simulink model "InductionHeating_bb_4"  (R2026b)
settings: Solver=FixedStepDiscrete  StopTime=0.008
PostLoadFcn:
  | Ts = 1e-6;Ts_fpga=10e-9;   R=3; Capa=300e-9;L=100e-6;Pejo_factor=1;
InitFcn:
  | Ts = 1e-6;Ts_fpga=10e-9;   R=3; Capa=300e-9;L=100e-6;Pejo_factor=1;
undefined symbols (not defined in the file or in its folder): DiscIntNeverNeededParam, ee_sli_rtmsupport, gcbh, isSetWhenUndefinedState, MATESOCwDio
libraries: fl_lib x67, nesl_utility x40, hdlsllib x32, simulink x15, eeGeneralControl x9, ee_lib x3
(part 6 of 7)

== system InductionHeating_bb_4/soc16/DynamicMultMAT/add2 ==
  E : Inport
  In1 : Inport  Port=2
  In2 : Inport  Port=3
  In4 : Inport  Port=4
  In5 : Inport  Port=5
  In7 : Inport  Port=6
  In8 : Inport  Port=7
  In10 : Inport  Port=8
  In11 : Inport  Port=9
  Add{3..6} (4 alike) : Sum
  Unit Delay Enabled Synchronous{1..3,22} (4 alike) : hdlsllib/Discrete/Unit Delay Enabled Synchronous  InitialCondition=0.0  SampleTime=-1
  y : Outport
  y1 : Outport  Port=2
  y2 : Outport  Port=3
  y3 : Outport  Port=4
  wires:
  In11/1 -> Add6/2
  In7/1 -> Add5/1
  Unit Delay Enabled Synchronous22/1 -> y/1
  Unit Delay Enabled Synchronous2/1 -> y2/1
  In10/1 -> Add6/1
  In2/1 -> Add3/2
  In8/1 -> Add5/2
  In4/1 -> Add4/1
  E/1 -> Unit Delay Enabled Synchronous22/2, Unit Delay Enabled Synchronous1/2, Unit Delay Enabled Synchronous2/2, Unit Delay Enabled Synchronous3/2
  Unit Delay Enabled Synchronous3/1 -> y3/1
  Unit Delay Enabled Synchronous1/1 -> y1/1
  Add5/1 -> Unit Delay Enabled Synchronous2/1
  Add3/1 -> Unit Delay Enabled Synchronous22/1
  Add6/1 -> Unit Delay Enabled Synchronous3/1
  In5/1 -> Add4/2
  In1/1 -> Add3/1
  Add4/1 -> Unit Delay Enabled Synchronous1/1

== system InductionHeating_bb_4/soc16/DynamicMultMAT/add3 ==
  E : Inport
  In1 : Inport  Port=2
  In2 : Inport  Port=3
  In4 : Inport  Port=4
  In5 : Inport  Port=5
  In7 : Inport  Port=6
  In8 : Inport  Port=7
  In10 : Inport  Port=8
  In11 : Inport  Port=9
  Add{3..6} (4 alike) : Sum
  Unit Delay Enabled Synchronous{1..3,22} (4 alike) : hdlsllib/Discrete/Unit Delay Enabled Synchronous  InitialCondition=0.0  SampleTime=-1
  y : Outport
  y1 : Outport  Port=2
  y2 : Outport  Port=3
  y3 : Outport  Port=4
  wires:
  Add4/1 -> Unit Delay Enabled Synchronous1/1
  In1/1 -> Add3/1
  In5/1 -> Add4/2
  Add6/1 -> Unit Delay Enabled Synchronous3/1
  Add3/1 -> Unit Delay Enabled Synchronous22/1
  Add5/1 -> Unit Delay Enabled Synchronous2/1
  Unit Delay Enabled Synchronous1/1 -> y1/1
  Unit Delay Enabled Synchronous3/1 -> y3/1
  E/1 -> Unit Delay Enabled Synchronous3/2, Unit Delay Enabled Synchronous2/2, Unit Delay Enabled Synchronous1/2, Unit Delay Enabled Synchronous22/2
  In4/1 -> Add4/1
  In8/1 -> Add5/2
  In2/1 -> Add3/2
  In10/1 -> Add6/1
  Unit Delay Enabled Synchronous2/1 -> y2/1
  Unit Delay Enabled Synchronous22/1 -> y/1
  In7/1 -> Add5/1
  In11/1 -> Add6/2

== system InductionHeating_bb_4/soc16/DynamicMultMAT/add4 ==
  E : Inport
  In1 : Inport  Port=2
  In2 : Inport  Port=3
  In4 : Inport  Port=4
  In5 : Inport  Port=5
  In7 : Inport  Port=6
  In8 : Inport  Port=7
  In10 : Inport  Port=8
  In11 : Inport  Port=9
  Add{3..6} (4 alike) : Sum
  Unit Delay Enabled Synchronous{1..3,22} (4 alike) : hdlsllib/Discrete/Unit Delay Enabled Synchronous  InitialCondition=0.0  SampleTime=-1
  y : Outport
  y1 : Outport  Port=2
  y2 : Outport  Port=3
  y3 : Outport  Port=4
  wires:
  In11/1 -> Add6/2
  In7/1 -> Add5/1
  Unit Delay Enabled Synchronous22/1 -> y/1
  Unit Delay Enabled Synchronous2/1 -> y2/1
  In10/1 -> Add6/1
  In2/1 -> Add3/2
  In8/1 -> Add5/2
  In4/1 -> Add4/1
  E/1 -> Unit Delay Enabled Synchronous22/2, Unit Delay Enabled Synchronous1/2, Unit Delay Enabled Synchronous2/2, Unit Delay Enabled Synchronous3/2
  Unit Delay Enabled Synchronous3/1 -> y3/1
  Unit Delay Enabled Synchronous1/1 -> y1/1
  Add5/1 -> Unit Delay Enabled Synchronous2/1
  Add3/1 -> Unit Delay Enabled Synchronous22/1
  Add6/1 -> Unit Delay Enabled Synchronous3/1
  In5/1 -> Add4/2
  In1/1 -> Add3/1
  Add4/1 -> Unit Delay Enabled Synchronous1/1

== system InductionHeating_bb_4/soc16/DynamicMultMAT/dot1 ==
  note: dot1
  In1 : Inport
  In2 : Inport  Port=2
  In3 : Inport  Port=3
  In4 : Inport  Port=4
  In5 : Inport  Port=5
  In6 : Inport  Port=6
  In7 : Inport  Port=7
  In8 : Inport  Port=8
  Dot Product{,1..3} (4 alike) : DotProduct  OutDataTypeStr=Inherit: Inherit via internal rule
  Out1 : Outport
  Out2 : Outport  Port=2
  Out3 : Outport  Port=3
  Out4 : Outport  Port=4
  wires:
  In1/1 -> Dot Product/2
  Dot Product/1 -> Out1/1
  In3/1 -> Dot Product1/2
  Dot Product1/1 -> Out2/1
  In2/1 -> Dot Product/1
  Dot Product3/1 -> Out4/1
  Dot Product2/1 -> Out3/1
  In7/1 -> Dot Product3/2
  In5/1 -> Dot Product2/2
  In8/1 -> Dot Product3/1
  In4/1 -> Dot Product1/1
  In6/1 -> Dot Product2/1

== system InductionHeating_bb_4/soc16/DynamicMultMAT/dot2 ==
  In1 : Inport
  y : Inport  Port=2
  In3 : Inport  Port=3
  y1 : Inport  Port=4
  In5 : Inport  Port=5
  y2 : Inport  Port=6
  In7 : Inport  Port=7
  y3 : Inport  Port=8
  Dot Product{4..7} (4 alike) : DotProduct  OutDataTypeStr=Inherit: Inherit via internal rule
  Out1 : Outport
  Out2 : Outport  Port=2
  Out3 : Outport  Port=3
  Out4 : Outport  Port=4
  wires:
  In3/1 -> Dot Product5/2
  Dot Product7/1 -> Out4/1
  Dot Product4/1 -> Out1/1
  Dot Product6/1 -> Out3/1
  In1/1 -> Dot Product4/2
  In7/1 -> Dot Product7/2
  Dot Product5/1 -> Out2/1
  In5/1 -> Dot Product6/2
  y/1 -> Dot Product4/1
  y1/1 -> Dot Product5/1
  y2/1 -> Dot Product6/1
  y3/1 -> Dot Product7/1

== system InductionHeating_bb_4/soc16/DynamicMultMAT/dot3 ==
  In1 : Inport
  y : Inport  Port=2
  In3 : Inport  Port=3
  y1 : Inport  Port=4
  In5 : Inport  Port=5
  y2 : Inport  Port=6
  In7 : Inport  Port=7
  y3 : Inport  Port=8
  Dot Product{8..11} (4 alike) : DotProduct  OutDataTypeStr=Inherit: Inherit via internal rule
  Out1 : Outport
  Out2 : Outport  Port=2
  Out3 : Outport  Port=3
  Out4 : Outport  Port=4
  wires:
  Dot Product11/1 -> Out4/1
  Dot Product10/1 -> Out3/1
  Dot Product8/1 -> Out1/1
  Dot Product9/1 -> Out2/1
  In3/1 -> Dot Product9/2
  In5/1 -> Dot Product10/2
  In7/1 -> Dot Product11/2
  In1/1 -> Dot Product8/2
  y3/1 -> Dot Product11/1
  y2/1 -> Dot Product10/1
  y/1 -> Dot Product8/1
  y1/1 -> Dot Product9/1

== system InductionHeating_bb_4/soc16/DynamicMultMAT/dot4 ==
  In1 : Inport
  In2 : Inport  Port=2
  In3 : Inport  Port=3
  In4 : Inport  Port=4
  In5 : Inport  Port=5
  Dot Product{12..15} (4 alike) : DotProduct  OutDataTypeStr=Inherit: Inherit via internal rule
  Out1 : Outport
  Out2 : Outport  Port=2
  Out3 : Outport  Port=3
  Out4 : Outport  Port=4
  wires:
  In1/1 -> Dot Product15/2, Dot Product14/2, Dot Product13/2, Dot Product12/2
  Dot Product14/1 -> Out3/1
  In5/1 -> Dot Product15/1
  In3/1 -> Dot Product13/1
  Dot Product15/1 -> Out4/1
  Dot Product13/1 -> Out2/1
  Dot Product12/1 -> Out1/1
  In2/1 -> Dot Product12/1
  In4/1 -> Dot Product14/1

== system InductionHeating_bb_4/soc16/DynamicMultMAT/mult1 ==
  In1 : Inport
  In2 : Inport  Port=2
  In3 : Inport  Port=3
  In4 : Inport  Port=4
  In5 : Inport  Port=5
  In6 : Inport  Port=6
  In7 : Inport  Port=7
  In8 : Inport  Port=8
  mullt{1..4} (4 alike) : Product
  DxCol*DxRow : Outport
  DxCol*DxRow1 : Outport  Port=2
  DxCol*DxRow2 : Outport  Port=3
  DxCol*DxRow3 : Outport  Port=4
  wires:
  mullt4/1 -> DxCol*DxRow3/1  "DxCol*DxRow"
  In2/1 -> mullt1/2
  In4/1 -> mullt2/2
  mullt2/1 -> DxCol*DxRow1/1  "DxCol*DxRow"
  In1/1 -> mullt1/1
  In8/1 -> mullt4/2
  In3/1 -> mullt2/1
  In6/1 -> mullt3/2
  In7/1 -> mullt4/1
  mullt1/1 -> DxCol*DxRow/1  "DxCol*DxRow"
  mullt3/1 -> DxCol*DxRow2/1  "DxCol*DxRow"
  In5/1 -> mullt3/1

== system InductionHeating_bb_4/soc16/DynamicMultMAT/mult2 ==
  In1 : Inport
  In2 : Inport  Port=2
  In3 : Inport  Port=3
  In4 : Inport  Port=4
  In5 : Inport  Port=5
  In6 : Inport  Port=6
  In7 : Inport  Port=7
  In8 : Inport  Port=8
  mullt{1..4} (4 alike) : Product
  DxCol*DxRow : Outport
  DxCol*DxRow1 : Outport  Port=2
  DxCol*DxRow2 : Outport  Port=3
  DxCol*DxRow3 : Outport  Port=4
  wires:
  In5/1 -> mullt3/1
  mullt3/1 -> DxCol*DxRow2/1  "DxCol*DxRow"
  mullt1/1 -> DxCol*DxRow/1  "DxCol*DxRow"
  In7/1 -> mullt4/1
  In6/1 -> mullt3/2
  In3/1 -> mullt2/1
  In8/1 -> mullt4/2
  In1/1 -> mullt1/1
  mullt2/1 -> DxCol*DxRow1/1  "DxCol*DxRow"
  In4/1 -> mullt2/2
  In2/1 -> mullt1/2
  mullt4/1 -> DxCol*DxRow3/1  "DxCol*DxRow"

== system InductionHeating_bb_4/soc16/DynamicMultMAT/mult3 ==
  In1 : Inport
  In2 : Inport  Port=2
  In3 : Inport  Port=3
  In4 : Inport  Port=4
  In5 : Inport  Port=5
  In6 : Inport  Port=6
  In7 : Inport  Port=7
  In8 : Inport  Port=8
  mullt{1..4} (4 alike) : Product
  DxCol*DxRow : Outport
  DxCol*DxRow1 : Outport  Port=2
  DxCol*DxRow2 : Outport  Port=3
  DxCol*DxRow3 : Outport  Port=4
  wires:
  mullt4/1 -> DxCol*DxRow3/1  "DxCol*DxRow"
  In2/1 -> mullt1/2
  In4/1 -> mullt2/2
  mullt2/1 -> DxCol*DxRow1/1  "DxCol*DxRow"
  In1/1 -> mullt1/1
  In8/1 -> mullt4/2
  In3/1 -> mullt2/1
  In6/1 -> mullt3/2
  In7/1 -> mullt4/1
  mullt1/1 -> DxCol*DxRow/1  "DxCol*DxRow"
  mullt3/1 -> DxCol*DxRow2/1  "DxCol*DxRow"
  In5/1 -> mullt3/1

== system InductionHeating_bb_4/soc16/DynamicMultMAT/mult4 ==
  In1 : Inport
  In2 : Inport  Port=2
  In3 : Inport  Port=3
  In4 : Inport  Port=4
  In5 : Inport  Port=5
  In6 : Inport  Port=6
  In7 : Inport  Port=7
  In8 : Inport  Port=8
  mullt{1..4} (4 alike) : Product
  DxCol*DxRow : Outport
  DxCol*DxRow1 : Outport  Port=2
  DxCol*DxRow2 : Outport  Port=3
  DxCol*DxRow3 : Outport  Port=4
  wires:
  In5/1 -> mullt3/1
  mullt3/1 -> DxCol*DxRow2/1  "DxCol*DxRow"
  mullt1/1 -> DxCol*DxRow/1  "DxCol*DxRow"
  In7/1 -> mullt4/1
  In6/1 -> mullt3/2
  In3/1 -> mullt2/1
  In8/1 -> mullt4/2
  In1/1 -> mullt1/1
  mullt2/1 -> DxCol*DxRow1/1  "DxCol*DxRow"
  In4/1 -> mullt2/2
  In2/1 -> mullt1/2
  mullt4/1 -> DxCol*DxRow3/1  "DxCol*DxRow"

== system InductionHeating_bb_4/soc16/DynamicMultMAT/multdiv1 ==
  In1 : Inport
  In2 : Inport  Port=2
  Demux : Demux  Outputs=[8 8]
  Divide5 : Product  Commented=on
  Mux : Mux  Inputs=2
  mmul8_1 : Subsystem
      mask help: To split one 1x8 vector multiplication
      mask Display: disp('1X8')
  mmul8_11 : Subsystem
      mask help: To split one 1x8 vector multiplication
      mask Display: disp('1X8')
  DxCol_ : Outport
  wires:
  In1/1 -> mmul8_1/1(In1), mmul8_11/1(In1), Divide5/1
  Demux/1 -> mmul8_11/2(In2)
  Demux/2 -> mmul8_1/2(In2)
  In2/1 -> Demux/1
  mmul8_11/1(Out1) -> Mux/1
  mmul8_1/1(Out1) -> Mux/2
  Mux/1 -> DxCol_/1

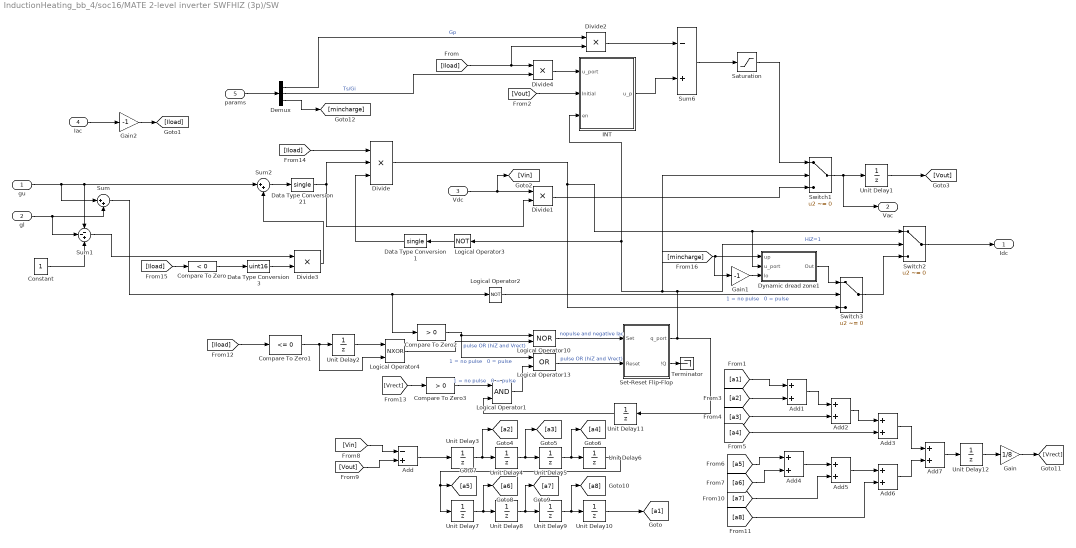
== system InductionHeating_bb_4/soc16/MATE 2-level inverter SWFHIZ (3p)/SW ==
  gu : Inport
  gl : Inport  Port=2
  Vdc : Inport  Port=3
  Iac : Inport  Port=4
  params : Inport  Port=5
  Add : Sum  Inputs=-+
  Add{1..7} (7 alike) : Sum  Inputs=2
  Compare To Zero : simulink/Logic and Bit Operations/Compare To Zero  relop=<  OutDataTypeStr=boolean
  Compare To Zero1 : simulink/Logic and Bit Operations/Compare To Zero  relop=<=  OutDataTypeStr=boolean
  Compare To Zero2 : simulink/Logic and Bit Operations/Compare To Zero  relop=>  OutDataTypeStr=boolean
  Compare To Zero3 : simulink/Logic and Bit Operations/Compare To Zero  relop=>  OutDataTypeStr=boolean
  Constant : Constant  OutDataTypeStr=uint16  SampleTime=Ts
  Data Type Conversion1 : DataTypeConversion  OutDataTypeStr=single  RndMeth=Nearest  SaturateOnIntegerOverflow=off
  Data Type Conversion21 : DataTypeConversion  OutDataTypeStr=single  RndMeth=Nearest  SaturateOnIntegerOverflow=off
  Data Type Conversion3 : DataTypeConversion  OutDataTypeStr=uint16  RndMeth=Nearest  SaturateOnIntegerOverflow=off
  Demux : Demux  Outputs=[1 1 1]
  Divide : Product  Inputs=3
  Divide{1..4} (4 alike) : Product
  Dynamic dread zone1 : Subsystem
  Gain : Gain  Gain=1/8
  Gain1 : Gain  Gain=-1
  Gain2 : Gain  Gain=-1
  INT : Subsystem
  Logical Operator1 : Logic  AllPortsSameDT=off  OutDataTypeStr=boolean
  Logical Operator10 : Logic  Operator=NOR  AllPortsSameDT=off  OutDataTypeStr=boolean
  Logical Operator13 : Logic  Operator=OR  AllPortsSameDT=off  OutDataTypeStr=boolean
  Logical Operator2 : Logic  Operator=NOT  AllPortsSameDT=off  OutDataTypeStr=boolean
  Logical Operator3 : Logic  Operator=NOT  AllPortsSameDT=off  OutDataTypeStr=boolean
  Logical Operator4 : Logic  Operator=NXOR  AllPortsSameDT=off  OutDataTypeStr=boolean
  Saturation : Saturate  UpperLimit=inf  LowerLimit=0
  Set-Reset Flip-Flop : Subsystem  AncestorBlock=eeGeneralControl/Set-Reset Flip-Flop  LoadFcn=ee_sli_rtmsupport( 'loadfcn', gcbh );  Variant=on  VariantControlMode=label  LabelModeActiveChoice=Discrete  mask(Set-Reset Flip-Flop){UndefState=Set, Q0=0, Ts=Ts}
      mask prompts: UndefState "physmod:ee:library:comments:control:eeGeneralControl:PriorityWhenUndefinedState_MP"; Q0 "physmod:ee:library:comments:control:eeGeneralControl:InitialConditionForQState_MP"; Ts "physmod:ee:library:comments:control:eeGeneralControl:SampleTime1ForInherited_MP"
      mask help: physmod:ee:library:comments:control:eeGeneralControl:SetResetFlipFlop_MD
      mask init:
      | [timeDomain,isSetWhenUndefinedState] = ee.mask.initializeSetResetFlipFlop(gcb,Q0,Ts,UndefState);%#ok
      settings: CopyFcn=ee_sli_rtmsupport( 'copyfcn', gcbh );  DeleteFcn=ee_sli_rtmsupport( 'deletefcn', gcbh );  ModelCloseFcn=ee_sli_rtmsupport( 'modelclosefcn', gcbh );  PostSaveFcn=ee_sli_rtmsupport( 'postsavefcn', gcbh );  PreCopyFcn=ee_sli_rtmsupport( 'precopyfcn', gcbh );  OpenFcn=ee_sli_rtmsupport( 'openfcn', gcbh );  CloseFcn=ee_sli_rtmsupport( 'closefcn', gcbh );  PreDeleteFcn=ee_sli_rtmsupport( 'predeletefcn', gcbh );
      mask Help: web(nesl_help(gcbh))
      mask TypeOptions UndefState: physmod:ee:library:comments:control:eeGeneralControl:Reset_PV | physmod:ee:library:comments:control:eeGeneralControl:Set_PV
      mask DialogControl ParameterGroupVar Prompt: physmod:ee:library:comments:control:eeGeneralControl:tab_Parameters
      mask DialogControl UndefState Prompt: Priority when undefined state
      mask DialogControl Q0 Prompt: Initial condition for Q state
      mask DialogControl Ts Prompt: Sample time (-1 for inherited)
      mask Display: ee.mask.drawSetResetFlipFlop;
  Sum : Sum  Inputs=|++
  Sum1 : Sum  Inputs=--+
  Sum2 : Sum  Inputs=|++
  Sum6 : Sum  Inputs=-+  InputSameDT=on  SaturateOnIntegerOverflow=on  SampleTime=Ts  OutDataTypeStr=Inherit: Same as first input
  Switch1 : Switch  Criteria=u2 ~= 0  SaturateOnIntegerOverflow=off  InputSameDT=off
  Switch2 : Switch  Criteria=u2 ~= 0  Threshold=0.5  SaturateOnIntegerOverflow=off  InputSameDT=off
  Switch3 : Switch  Criteria=u2 ~= 0  Threshold=0.5  SaturateOnIntegerOverflow=off  InputSameDT=off
  Terminator : Terminator
  Unit Delay{1..12} (12 alike) : UnitDelay  SampleTime=Ts
  Idc : Outport  VectorParamsAs1DForOutWhenUnconnected=off
  Vac : Outport  Port=2  VectorParamsAs1DForOutWhenUnconnected=off
  wires:
  Set-Reset Flip-Flop/2(!Q) -> Terminator/1
  Iac/1 -> Gain2/1
  Set-Reset Flip-Flop/1(q_port) -> Logical Operator3/1, INT/3(en), Switch1/2, Switch2/2, Unit Delay11/1  "HiZ=1"
  Sum6/1 -> Saturation/1
  Switch1/1 -> Unit Delay1/1, Vac/1
  Constant/1 -> Sum1/3
  gl/1 -> Sum1/2, Sum/2
  Logical Operator3/1 -> Data Type Conversion1/1
  Logical Operator2/1 -> Switch3/2  "1 = no pulse   0 = pulse"
  Vdc/1 -> Divide1/1, [Vin]
  Sum/1 -> Logical Operator2/1, Compare To Zero2/1
  gu/1 -> Sum/1, Sum2/1, Sum1/1
  Sum2/1 -> Data Type Conversion21/1
  Divide1/1 -> Switch1/3
  Saturation/1 -> Switch1/1
  Switch2/1 -> Idc/1
  Divide/1 -> Switch3/3, Dynamic dread zone1/2(u_port), Switch2/1
  Dynamic dread zone1/1(Out) -> Switch3/1
  Switch3/1 -> Switch2/3
  Unit Delay1/1 -> [Vout]
  Logical Operator10/1 -> Set-Reset Flip-Flop/1(Set)  "nopulse and negative Iac"
  [Vout] -> INT/2(Initial)
  [Vin] -> Add/1
  [Vout] -> Add/2
  Add/1 -> Unit Delay3/1
  Unit Delay3/1 -> [a2], Unit Delay4/1
  Unit Delay4/1 -> [a3], Unit Delay5/1
  Unit Delay5/1 -> [a4], Unit Delay6/1
  Unit Delay6/1 -> [a5], Unit Delay7/1
  Unit Delay7/1 -> [a6], Unit Delay8/1
  Unit Delay8/1 -> [a7], Unit Delay9/1
  Unit Delay9/1 -> Unit Delay10/1, [a8]
  [a4] -> Add3/2
  [a3] -> Add2/2
  [a2] -> Add1/2
  [a1] -> Add1/1
  Compare To Zero1/1 -> Logical Operator4/2, Unit Delay2/1
  INT/1(u_p) -> Sum6/2
  [Vrect] -> Compare To Zero3/1
  Unit Delay11/1 -> Logical Operator1/2
  Logical Operator13/1 -> Set-Reset Flip-Flop/2(Reset)  "pulse OR (hiZ and Vrect)"
  Logical Operator1/1 -> Logical Operator13/2
  [Iload] -> Divide4/1, Divide2/2
  [Iload] -> Divide/1
  [Iload] -> Compare To Zero/1
  Compare To Zero/1 -> Data Type Conversion3/1
  Sum1/1 -> Divide3/1
  Gain2/1 -> [Iload]
  Demux/1 -> Divide2/1  "Gp"
  Divide2/1 -> Sum6/1
  Divide4/1 -> INT/1(u_port)
  Demux/2 -> Divide4/2  "Ts/Gi"
  Demux/3 -> [mincharge]
  [mincharge] -> Dynamic dread zone1/1(up), Gain1/1
  Gain1/1 -> Dynamic dread zone1/3(lo)
  params/1 -> Demux/1
  Data Type Conversion21/1 -> Divide1/2, Divide/2
  Data Type Conversion1/1 -> Divide/3
  Gain/1 -> [Vrect]
  [a5] -> Add4/1
  [a6] -> Add4/2
  [a7] -> Add5/2
  [a8] -> Add6/2
  Add1/1 -> Add2/1
  Add2/1 -> Add3/1
  Add4/1 -> Add5/1
  Add5/1 -> Add6/1
  Add3/1 -> Add7/1
  Add6/1 -> Add7/2
  Add7/1 -> Unit Delay12/1
  Divide3/1 -> Sum2/2
  Data Type Conversion3/1 -> Divide3/2
  Unit Delay2/1 -> Logical Operator4/1
  Logical Operator4/1 -> Logical Operator10/2  "pulse OR (hiZ and Vrect)"
  Compare To Zero2/1 -> Logical Operator10/1, Logical Operator13/1  "1 = no pulse   0 = pulse"
  Unit Delay10/1 -> [a1]
  Compare To Zero3/1 -> Logical Operator1/1  "1 = no pulse   0 = pulse"
  [Iload] -> Compare To Zero1/1
  Unit Delay12/1 -> Gain/1

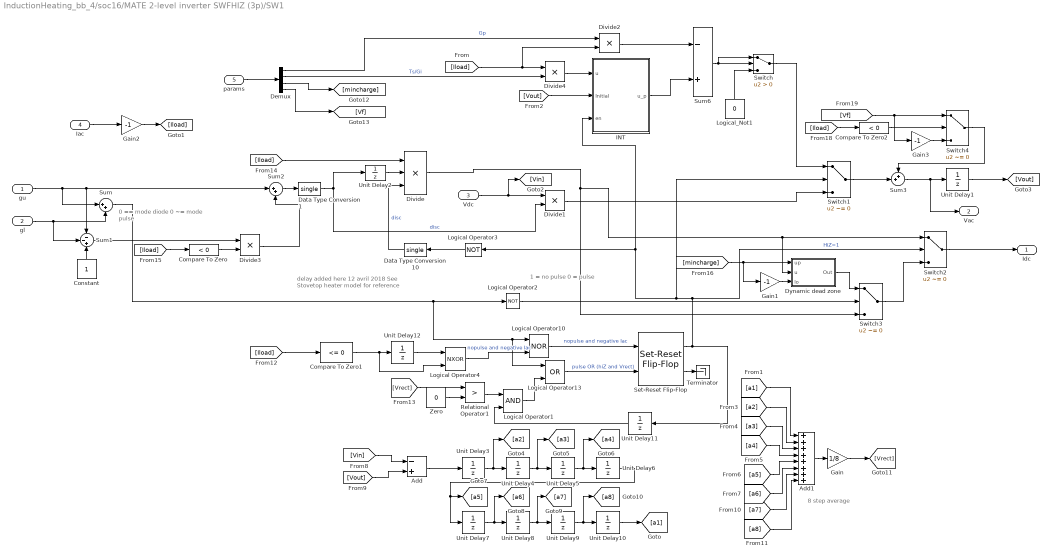
== system InductionHeating_bb_4/soc16/MATE 2-level inverter SWFHIZ (3p)/SW1 ==
  note: 8 step average
  note: 1 = no pulse
      | 0 = pulse
  note: 0 == mode diode
      | 0 ~= mode pulse
  note: delay added here 12 avril 2018
      | See Stovetop heater model for reference
  gu : Inport
  gl : Inport  Port=2
  Vdc : Inport  Port=3
  Iac : Inport  Port=4
  params : Inport  Port=5
  Add : Sum  Inputs=-+
  Add1 : Sum  Inputs=8
  Compare To Zero : simulink/Logic and Bit Operations/Compare To Zero  relop=<  OutDataTypeStr=boolean
  Compare To Zero1 : simulink/Logic and Bit Operations/Compare To Zero  relop=<=  OutDataTypeStr=boolean
  Compare To Zero2 : simulink/Logic and Bit Operations/Compare To Zero  relop=<  OutDataTypeStr=boolean
  Constant : Constant  OutDataTypeStr=uint16
  Data Type Conversion1 : DataTypeConversion  OutDataTypeStr=single  RndMeth=Nearest  SaturateOnIntegerOverflow=off
  Data Type Conversion10 : DataTypeConversion  OutDataTypeStr=single  RndMeth=Nearest  SaturateOnIntegerOverflow=off
  Demux : Demux
  Divide : Product  Inputs=3
  Divide{1..4} (4 alike) : Product
  Dynamic dead zone : Subsystem
  Gain : Gain  Gain=1/8
  Gain1 : Gain  Gain=-1
  Gain2 : Gain  Gain=-1
  Gain3 : Gain  Gain=-1
  INT : Subsystem
  Logical Operator1 : Logic  AllPortsSameDT=off  OutDataTypeStr=boolean
  Logical Operator10 : Logic  Operator=NOR  AllPortsSameDT=off  OutDataTypeStr=boolean
  Logical Operator13 : Logic  Operator=OR  AllPortsSameDT=off  OutDataTypeStr=boolean
  Logical Operator2 : Logic  Operator=NOT  AllPortsSameDT=off  OutDataTypeStr=boolean
  Logical Operator3 : Logic  Operator=NOT  AllPortsSameDT=off  OutDataTypeStr=boolean
  Logical Operator4 : Logic  Operator=NXOR  AllPortsSameDT=off  OutDataTypeStr=boolean
  Logical_Not1 : Constant  Value=0  OutDataTypeStr=single  SampleTime=-1
  Relational Operator1 : RelationalOperator  Operator=>  OutDataTypeStr=boolean  InputSameDT=off
  Set-Reset Flip-Flop : eeGeneralControl/Set-Reset Flip-Flop  LabelModeActiveChoice=Discrete  UndefState=Set  Q0=0  Ts=Ts
  Sum : Sum  Inputs=|++
  Sum1 : Sum  Inputs=--+
  Sum2 : Sum  Inputs=|++
  Sum3 : Sum  Inputs=++|
  Sum6 : Sum  Inputs=-+  InputSameDT=on  SaturateOnIntegerOverflow=on  SampleTime=Ts  OutDataTypeStr=Inherit: Same as first input
  Switch : Switch  Criteria=u2 > Threshold  SaturateOnIntegerOverflow=off  InputSameDT=off
  Switch1 : Switch  Criteria=u2 ~= 0  SaturateOnIntegerOverflow=off  InputSameDT=off
  Switch2 : Switch  Criteria=u2 ~= 0  Threshold=0.5  SaturateOnIntegerOverflow=off  InputSameDT=off
  Switch3 : Switch  Criteria=u2 ~= 0  Threshold=0.5  SaturateOnIntegerOverflow=off  InputSameDT=off
  Switch4 : Switch  Criteria=u2 ~= 0  Threshold=0.5  SaturateOnIntegerOverflow=off  InputSameDT=off
  Terminator : Terminator
  Unit Delay{1..12} (12 alike) : UnitDelay  SampleTime=Ts
  Zero : Constant  Value=0  OutDataTypeStr=single
  Idc : Outport  VectorParamsAs1DForOutWhenUnconnected=off
  Vac : Outport  Port=2  VectorParamsAs1DForOutWhenUnconnected=off
  wires:
  Logical Operator4/1 -> Logical Operator10/2  "nopulse and negative Iac"
  Unit Delay12/1 -> Logical Operator4/1
  Unit Delay10/1 -> [a1]
  Unit Delay2/1 -> Divide/2
  Switch4/1 -> Sum3/1
  Gain3/1 -> Switch4/3
  [Vf] -> Switch4/1, Gain3/1
  Compare To Zero2/1 -> Switch4/2
  Sum3/1 -> Vac/1, Unit Delay1/1
  [Iload] -> Compare To Zero2/1
  Demux/4 -> [Vf]
  params/1 -> Demux/1
  Gain1/1 -> Dynamic dead zone/3(lo)
  [mincharge] -> Gain1/1, Dynamic dead zone/1(up)
  Demux/3 -> [mincharge]
  Demux/2 -> Divide4/2  "Ts/Gi"
  Divide4/1 -> INT/1(u)
  Divide2/1 -> Sum6/1
  Demux/1 -> Divide2/1  "Gp"
  Gain2/1 -> [Iload]
  Sum1/1 -> Divide3/1
  Compare To Zero/1 -> Divide3/2
  [Iload] -> Compare To Zero/1
  [Iload] -> Divide/1
  [Iload] -> Divide2/2, Divide4/1
  Logical Operator1/1 -> Logical Operator13/2
  Logical Operator13/1 -> Set-Reset Flip-Flop/2  "pulse OR (hiZ and Vrect)"
  Unit Delay11/1 -> Logical Operator1/2
  Relational Operator1/1 -> Logical Operator1/1
  Zero/1 -> Relational Operator1/2
  [Vrect] -> Relational Operator1/1
  INT/1(u_p) -> Sum6/2
  Compare To Zero1/1 -> Unit Delay12/1, Logical Operator4/2
  [Iload] -> Compare To Zero1/1
  Gain/1 -> [Vrect]
  Add1/1 -> Gain/1
  [a1] -> Add1/1
  [a8] -> Add1/8
  [a2] -> Add1/2
  [a7] -> Add1/7
  [a6] -> Add1/6
  [a3] -> Add1/3
  [a5] -> Add1/5
  [a4] -> Add1/4
  Unit Delay9/1 -> Unit Delay10/1, [a8]
  Unit Delay8/1 -> Unit Delay9/1, [a7]
  Unit Delay7/1 -> Unit Delay8/1, [a6]
  Unit Delay6/1 -> Unit Delay7/1, [a5]
  Unit Delay5/1 -> Unit Delay6/1, [a4]
  Unit Delay4/1 -> Unit Delay5/1, [a3]
  Unit Delay3/1 -> Unit Delay4/1, [a2]
  Add/1 -> Unit Delay3/1
  [Vout] -> Add/2
  [Vin] -> Add/1
  [Vout] -> INT/2(Initial)
  Logical Operator10/1 -> Set-Reset Flip-Flop/1  "nopulse and negative Iac"
  Unit Delay1/1 -> [Vout]
  Switch3/1 -> Switch2/3
  Dynamic dead zone/1(Out) -> Switch3/1
  Divide/1 -> Switch2/1, Dynamic dead zone/2(u), Switch3/3
  Switch2/1 -> Idc/1
  Switch/1 -> Switch1/1
  Divide1/1 -> Switch1/3
  Sum2/1 -> Data Type Conversion1/1
  gu/1 -> Sum1/1, Sum2/1, Sum/1
  Sum/1 -> Logical Operator2/1, Logical Operator10/1, Logical Operator13/1
  Vdc/1 -> [Vin], Divide1/1
  Logical Operator2/1 -> Switch3/2
  Logical Operator3/1 -> Data Type Conversion10/1
  gl/1 -> Sum/2, Sum1/2
  Constant/1 -> Sum1/3
  Divide3/1 -> Sum2/2
  Switch1/1 -> Sum3/2
  Sum6/1 -> Switch/2, Switch/1
  Logical_Not1/1 -> Switch/3
  Set-Reset Flip-Flop/1 -> Unit Delay11/1, Switch2/2, Switch1/2, INT/3(en), Logical Operator3/1  "HiZ=1"
  Iac/1 -> Gain2/1
  Set-Reset Flip-Flop/2 -> Terminator/1
  Data Type Conversion10/1 -> Divide/3  "disc"
  Data Type Conversion1/1 -> Unit Delay2/1, Divide1/2  "disc"

== system InductionHeating_bb_4/soc16/PWM_Generator at Ts/PWM generator ==
  steps : Inport
  stepON : Inport  Port=2
  Add : Sum  Inputs=+-  OutDataTypeStr=int32
  Add1 : Sum  Inputs=+-  OutDataTypeStr=int32
  Constat : Constant  Value=0  OutDataTypeStr=int32  SampleTime=Ts
  Constat1 : Constant  OutDataTypeStr=int32  SampleTime=Ts
  Constat2 : Constant  Value=0  OutDataTypeStr=int32  SampleTime=Ts
  Constat3 : Constant  OutDataTypeStr=int32  SampleTime=Ts
  Data Type Conversion1 : DataTypeConversion  OutDataTypeStr=int32  RndMeth=Nearest  SaturateOnIntegerOverflow=off
  Data Type Conversion2 : DataTypeConversion  OutDataTypeStr=int32  RndMeth=Nearest  SaturateOnIntegerOverflow=off
  Logical Operator : Logic  AllPortsSameDT=off  OutDataTypeStr=boolean
  Relational Operator2 : RelationalOperator  OutDataTypeStr=boolean
  Relational Operator3 : RelationalOperator  OutDataTypeStr=boolean
  Relational Operator4 : RelationalOperator  Operator=<=  OutDataTypeStr=boolean
  Shift Arithmetic1 : ArithShift  BitShiftNumber=1  BitShiftDirection=Right
  Sum2 : Sum  InputSameDT=on  SaturateOnIntegerOverflow=on  OutDataTypeStr=Inherit: Same as first input
  Switch : Switch  Criteria=u2 ~= 0
  Switch1 : Switch  Criteria=u2 ~= 0
  Unit Delay Enabled Synchronous : hdlsllib/Discrete/Unit Delay Enabled Synchronous  InitialCondition=0.0  SampleTime=Ts
  Unit Delay Enabled Synchronous1 : hdlsllib/Discrete/Unit Delay Enabled Synchronous  InitialCondition=0.0  SampleTime=Ts
  Unit Delay1 : UnitDelay  SampleTime=Ts
  pulse : Outport  InitialOutput=0  VectorParamsAs1DForOutWhenUnconnected=off
  wires:
  Constat/1 -> Switch/1
  Switch/1 -> Sum2/1
  Unit Delay1/1 -> Relational Operator3/1, Switch1/3
  Sum2/1 -> Relational Operator4/1, Relational Operator2/1, Unit Delay1/1
  Data Type Conversion1/1 -> Add1/1
  Relational Operator3/1 -> Switch/2, Unit Delay Enabled Synchronous/2, Unit Delay Enabled Synchronous1/2, Switch1/2
  Data Type Conversion2/1 -> Shift Arithmetic1/1
  Constat1/1 -> Switch/3
  Relational Operator2/1 -> Logical Operator/1
  Relational Operator4/1 -> Logical Operator/2
  Logical Operator/1 -> pulse/1
  Add/1 -> Relational Operator4/2
  Constat2/1 -> Switch1/1
  Switch1/1 -> Sum2/2
  Shift Arithmetic1/1 -> Add/2, Relational Operator2/2
  steps/1 -> Unit Delay Enabled Synchronous/1
  stepON/1 -> Unit Delay Enabled Synchronous1/1
  Unit Delay Enabled Synchronous/1 -> Data Type Conversion1/1
  Unit Delay Enabled Synchronous1/1 -> Data Type Conversion2/1
  Add1/1 -> Relational Operator3/2, Add/1
  Constat3/1 -> Add1/2

== system InductionHeating_bb_4/soc16/PWM_Generator at Ts1/PWM generator ==
  steps : Inport
  stepON : Inport  Port=2
  Add : Sum  Inputs=+-  OutDataTypeStr=int32
  Add1 : Sum  Inputs=+-  OutDataTypeStr=int32
  Constat : Constant  Value=0  OutDataTypeStr=int32  SampleTime=Ts
  Constat1 : Constant  OutDataTypeStr=int32  SampleTime=Ts
  Constat2 : Constant  Value=0  OutDataTypeStr=int32  SampleTime=Ts
  Constat3 : Constant  OutDataTypeStr=int32  SampleTime=Ts
  Data Type Conversion1 : DataTypeConversion  OutDataTypeStr=int32  RndMeth=Nearest  SaturateOnIntegerOverflow=off
  Data Type Conversion2 : DataTypeConversion  OutDataTypeStr=int32  RndMeth=Nearest  SaturateOnIntegerOverflow=off
  Logical Operator : Logic  AllPortsSameDT=off  OutDataTypeStr=boolean
  Relational Operator2 : RelationalOperator  OutDataTypeStr=boolean
  Relational Operator3 : RelationalOperator  OutDataTypeStr=boolean
  Relational Operator4 : RelationalOperator  Operator=<=  OutDataTypeStr=boolean
  Shift Arithmetic1 : ArithShift  BitShiftNumber=1  BitShiftDirection=Right
  Sum2 : Sum  InputSameDT=on  SaturateOnIntegerOverflow=on  OutDataTypeStr=Inherit: Same as first input
  Switch : Switch  Criteria=u2 ~= 0
  Switch1 : Switch  Criteria=u2 ~= 0
  Unit Delay Enabled Synchronous : hdlsllib/Discrete/Unit Delay Enabled Synchronous  InitialCondition=0.0  SampleTime=Ts
  Unit Delay Enabled Synchronous1 : hdlsllib/Discrete/Unit Delay Enabled Synchronous  InitialCondition=0.0  SampleTime=Ts
  Unit Delay1 : UnitDelay  SampleTime=Ts
  pulse : Outport  InitialOutput=0  VectorParamsAs1DForOutWhenUnconnected=off
  wires:
  Constat3/1 -> Add1/2
  Add1/1 -> Add/1, Relational Operator3/2
  Unit Delay Enabled Synchronous1/1 -> Data Type Conversion2/1
  Unit Delay Enabled Synchronous/1 -> Data Type Conversion1/1
  stepON/1 -> Unit Delay Enabled Synchronous1/1
  steps/1 -> Unit Delay Enabled Synchronous/1
  Shift Arithmetic1/1 -> Relational Operator2/2, Add/2
  Switch1/1 -> Sum2/2
  Constat2/1 -> Switch1/1
  Add/1 -> Relational Operator4/2
  Logical Operator/1 -> pulse/1
  Relational Operator4/1 -> Logical Operator/2
  Relational Operator2/1 -> Logical Operator/1
  Constat1/1 -> Switch/3
  Data Type Conversion2/1 -> Shift Arithmetic1/1
  Relational Operator3/1 -> Switch1/2, Unit Delay Enabled Synchronous1/2, Unit Delay Enabled Synchronous/2, Switch/2
  Data Type Conversion1/1 -> Add1/1
  Sum2/1 -> Unit Delay1/1, Relational Operator2/1, Relational Operator4/1
  Unit Delay1/1 -> Switch1/3, Relational Operator3/1
  Switch/1 -> Sum2/1
  Constat/1 -> Switch/1

== system InductionHeating_bb_4/soc16/PWM_Generator at Ts2/PWM generator ==
  steps : Inport
  stepON : Inport  Port=2
  Add : Sum  Inputs=+-  OutDataTypeStr=int32
  Add1 : Sum  Inputs=+-  OutDataTypeStr=int32
  Constat : Constant  Value=0  OutDataTypeStr=int32  SampleTime=Ts
  Constat1 : Constant  OutDataTypeStr=int32  SampleTime=Ts
  Constat2 : Constant  Value=0  OutDataTypeStr=int32  SampleTime=Ts
  Constat3 : Constant  OutDataTypeStr=int32  SampleTime=Ts
  Data Type Conversion1 : DataTypeConversion  OutDataTypeStr=int32  RndMeth=Nearest  SaturateOnIntegerOverflow=off
  Data Type Conversion2 : DataTypeConversion  OutDataTypeStr=int32  RndMeth=Nearest  SaturateOnIntegerOverflow=off
  Logical Operator : Logic  AllPortsSameDT=off  OutDataTypeStr=boolean
  Relational Operator2 : RelationalOperator  OutDataTypeStr=boolean
  Relational Operator3 : RelationalOperator  OutDataTypeStr=boolean
  Relational Operator4 : RelationalOperator  Operator=<=  OutDataTypeStr=boolean
  Shift Arithmetic1 : ArithShift  BitShiftNumber=1  BitShiftDirection=Right
  Sum2 : Sum  InputSameDT=on  SaturateOnIntegerOverflow=on  OutDataTypeStr=Inherit: Same as first input
  Switch : Switch  Criteria=u2 ~= 0
  Switch1 : Switch  Criteria=u2 ~= 0
  Unit Delay Enabled Synchronous : hdlsllib/Discrete/Unit Delay Enabled Synchronous  InitialCondition=0.0  SampleTime=Ts
  Unit Delay Enabled Synchronous1 : hdlsllib/Discrete/Unit Delay Enabled Synchronous  InitialCondition=0.0  SampleTime=Ts
  Unit Delay1 : UnitDelay  SampleTime=Ts
  pulse : Outport  InitialOutput=0  VectorParamsAs1DForOutWhenUnconnected=off
  wires:
  Constat/1 -> Switch/1
  Switch/1 -> Sum2/1
  Unit Delay1/1 -> Relational Operator3/1, Switch1/3
  Sum2/1 -> Relational Operator4/1, Relational Operator2/1, Unit Delay1/1
  Data Type Conversion1/1 -> Add1/1
  Relational Operator3/1 -> Switch/2, Unit Delay Enabled Synchronous/2, Unit Delay Enabled Synchronous1/2, Switch1/2
  Data Type Conversion2/1 -> Shift Arithmetic1/1
  Constat1/1 -> Switch/3
  Relational Operator2/1 -> Logical Operator/1
  Relational Operator4/1 -> Logical Operator/2
  Logical Operator/1 -> pulse/1
  Add/1 -> Relational Operator4/2
  Constat2/1 -> Switch1/1
  Switch1/1 -> Sum2/2
  Shift Arithmetic1/1 -> Add/2, Relational Operator2/2
  steps/1 -> Unit Delay Enabled Synchronous/1
  stepON/1 -> Unit Delay Enabled Synchronous1/1
  Unit Delay Enabled Synchronous/1 -> Data Type Conversion1/1
  Unit Delay Enabled Synchronous1/1 -> Data Type Conversion2/1
  Add1/1 -> Relational Operator3/2, Add/1
  Constat3/1 -> Add1/2

== system InductionHeating_bb_4/soc16/RLCsw8/Diode2 ==
  Pejovic L-C-switch component : Subsystem  AncestorBlock=simetranss/FPGA/Pejovic L-C-switch component  mask(Pejovic Element for FPGA simulation){typ=Switch, Lon=LON, L=1, C=1, traprule=off, otherSW='coming soon', Ts=Ts, pcbp=off, showV=on, showI=on}
      mask prompts: typ "Element type"; Lon "Switch equivalent ON inductance (H)"; L "Inductor inductance (H)"; C "Capacitor capacitance (F)"; traprule "Use Trapezoidal rule (LC only)"; otherSW "Linked Compensated switch name"; Ts "Sample Time (s)"; pcbp "Precharge bypass (inverter only)"; showV "Show voltage port"; showI "Show current port"
      mask help:
      | Pejovic L-C-Switch element  in SimScape
      |
      | Implements either  an inductor, a capacitor or a switch using the Pejovic constant admittance method.
      |
      | For the Switch option, the user only has to select the equivalent ON-state inductance of the model, the corresponding Capacitance is computed internally. In the Pejovic model, Ts/Lon=Coff/Ts (Backward Euler) resulting in a constant admittance for the DAE solver.
      |
      |
      | Input signals;
      |
      | gate: the switch gate value (1 for ON , 0 for OFF) (with Switch option)
      mask init: same as InductionHeating_bb_4/MATEwDiode/Diode1/Pejovic L-C-switch component
      mask TypeOptions typ: Switch | Inductor | Capacitor | 2-level inverter switch
      mask Display:
      | plot(s1,s2,s3,s4,r1,r2,l1,l2,c1,c2,c3,c4,x1,x2,x3,x4);
      | color('blue')
      | port_label('LConn',1,'+')
      | disp([qq  10 10])
  Relational Operator : RelationalOperator  Operator=>  OutDataTypeStr=boolean  RndMeth=Simplest  InputSameDT=off
  Relational Operator1 : RelationalOperator  Operator=>  OutDataTypeStr=boolean  RndMeth=Simplest  InputSameDT=off
  Resistor1 : fl_lib/Electrical/Electrical Elements/Resistor  R=RON Ohm  i_specify=off  i_priority=None  i=0 A  i_nominal_specify=off  i_nominal_value=1  i_nominal_unit=A  v_specify=off  v_priority=None  v=0 V  v_nominal_specify=off  v_nominal_value=1  v_nominal_unit=V
  Set-Reset Flip-Flop : eeGeneralControl/Set-Reset Flip-Flop  LabelModeActiveChoice=Discrete  UndefState=Set  Q0=0  Ts=Ts
  Terminator : Terminator
  Unit Delay : UnitDelay  SampleTime=Ts
  Vf : Constant  Value=0  SampleTime=Ts
  Vf2 : Constant  Value=VF  SampleTime=Ts
  currrent OFF : Constant  Value=0  SampleTime=Ts
  +V : PMIOPort  Side=Left
  -V : PMIOPort  Port=2  Side=Right
  wires:
  ? -> Relational Operator/1
  ? -> Relational Operator1/1
  Vf/1 -> Relational Operator/2
  Set-Reset Flip-Flop/2 -> Terminator/1
  currrent OFF/1 -> Relational Operator1/2
  Relational Operator1/1 -> Set-Reset Flip-Flop/2
  Unit Delay/1 -> Pejovic L-C-switch component/1(gate)
  Set-Reset Flip-Flop/1 -> Unit Delay/1
  Relational Operator/1 -> Set-Reset Flip-Flop/1
  Vf2/1 -> Pejovic L-C-switch component/2(Vf)
  connections:
  Resistor1/LConn1 -- Pejovic L-C-switch component/LConn1
  Pejovic L-C-switch component/RConn1 -- -V/RConn1
  Resistor1/RConn1 -- +V/RConn1

== system InductionHeating_bb_4/soc16/RLCsw8/Subsystem1 ==
  note: this 1/z adds one step of ~Q=0 if we want more than 1 step to refactorize everything
  trig : Inport
  trig1 : Inport  Port=2
  Logical Operator : Logic  Inputs=4  AllPortsSameDT=off  OutDataTypeStr=boolean
  Logical Operator1 : Logic  Operator=OR  AllPortsSameDT=off  OutDataTypeStr=boolean
  Relational Operator1 : RelationalOperator  Operator=~=  OutDataTypeStr=boolean  RndMeth=Simplest  InputSameDT=off
  Relational Operator2 : RelationalOperator  Operator=~=  OutDataTypeStr=boolean  RndMeth=Simplest  InputSameDT=off
  Scope : Scope  NumInputPorts=2
      settings: ActiveDisplayYMinimum=-1  ActiveDisplayYMaximum=1
  Set-Reset Flip-Flop : eeGeneralControl/Set-Reset Flip-Flop  LabelModeActiveChoice=Discrete  UndefState=Reset  Q0=0  Ts=Ts
      settings: LibrarySourceBlock=ee_sl_lib/General Control/Set-Reset Flip-Flop
  Unit Delay{,1..6} (7 alike) : UnitDelay  SampleTime=Ts
  q_port : Outport
  !Q : Outport  Port=2
  wires:
  Unit Delay1/1 -> Unit Delay2/1, Logical Operator/2
  Logical Operator/1 -> Scope/2, Set-Reset Flip-Flop/1
  Set-Reset Flip-Flop/1 -> Scope/1, q_port/1, Unit Delay3/1
  trig/1 -> Unit Delay/1, Relational Operator2/1
  Set-Reset Flip-Flop/2 -> !Q/1, Unit Delay4/1
  Unit Delay/1 -> Relational Operator2/2
  Unit Delay3/1 -> Unit Delay6/1
  Unit Delay4/1 -> Logical Operator/1, Unit Delay1/1
  Unit Delay5/1 -> Relational Operator1/2
  trig1/1 -> Relational Operator1/1, Unit Delay5/1
  Relational Operator2/1 -> Logical Operator1/1
  Relational Operator1/1 -> Logical Operator1/2
  Unit Delay2/1 -> Logical Operator/3
  Logical Operator1/1 -> Logical Operator/4
  Unit Delay6/1 -> Set-Reset Flip-Flop/2

== system InductionHeating_bb_4/soc16/RLCsw8/add8_1 ==
  In1 : Inport
  In2 : Inport  Port=2
  Add{1..8} (8 alike) : Sum  Inputs=2
  Demux2 : Demux  Outputs=8
  Demux3 : Demux  Outputs=8
  Mux2 : Mux  Inputs=8
  Out1 : Outport
  wires:
  Mux2/1 -> Out1/1
  In1/1 -> Demux2/1
  Demux3/6 -> Add6/2
  Demux3/8 -> Add8/2
  Demux2/5 -> Add5/1
  Demux2/7 -> Add7/1
  Demux2/4 -> Add4/1
  Demux3/5 -> Add5/2
  Demux2/6 -> Add6/1
  Add8/1 -> Mux2/8
  Add4/1 -> Mux2/4
  Add7/1 -> Mux2/7
  Add1/1 -> Mux2/2
  Add6/1 -> Mux2/6
  Demux2/3 -> Add3/1
  Demux3/2 -> Add1/2
  Demux2/8 -> Add8/1
  Demux2/1 -> Add2/1
  Demux2/2 -> Add1/1
  Demux3/1 -> Add2/2
  In2/1 -> Demux3/1
  Add2/1 -> Mux2/1
  Demux3/7 -> Add7/2
  Add5/1 -> Mux2/5
  Add3/1 -> Mux2/3
  Demux3/4 -> Add4/2
  Demux3/3 -> Add3/2

== system InductionHeating_bb_4/soc16/RLCsw8/add8_2 ==
  In1 : Inport
  In2 : Inport  Port=2
  Add{1..8} (8 alike) : Sum  Inputs=2
  Demux2 : Demux  Outputs=8
  Demux3 : Demux  Outputs=8
  Mux2 : Mux  Inputs=8
  Out1 : Outport
  wires:
  Demux3/3 -> Add3/2
  Demux3/4 -> Add4/2
  Add3/1 -> Mux2/3
  Add5/1 -> Mux2/5
  Demux3/7 -> Add7/2
  Add2/1 -> Mux2/1
  In2/1 -> Demux3/1
  Demux3/1 -> Add2/2
  Demux2/2 -> Add1/1
  Demux2/1 -> Add2/1
  Demux2/8 -> Add8/1
  Demux3/2 -> Add1/2
  Demux2/3 -> Add3/1
  Add6/1 -> Mux2/6
  Add1/1 -> Mux2/2
  Add7/1 -> Mux2/7
  Add4/1 -> Mux2/4
  Add8/1 -> Mux2/8
  Demux2/6 -> Add6/1
  Demux3/5 -> Add5/2
  Demux2/4 -> Add4/1
  Demux2/7 -> Add7/1
  Demux2/5 -> Add5/1
  Demux3/8 -> Add8/2
  Demux3/6 -> Add6/2
  In1/1 -> Demux2/1
  Mux2/1 -> Out1/1

== system InductionHeating_bb_4/soc16/RLCsw8/add8_3 ==
  In1 : Inport
  In2 : Inport  Port=2
  Add{1..8} (8 alike) : Sum  Inputs=2
  Demux2 : Demux  Outputs=8
  Demux3 : Demux  Outputs=8
  Mux2 : Mux  Inputs=8
  Out1 : Outport
  wires:
  Demux3/3 -> Add3/2
  Demux3/4 -> Add4/2
  Add3/1 -> Mux2/3
  Add5/1 -> Mux2/5
  Demux3/7 -> Add7/2
  Add2/1 -> Mux2/1
  In2/1 -> Demux3/1
  Demux3/1 -> Add2/2
  Demux2/2 -> Add1/1
  Demux2/1 -> Add2/1
  Demux2/8 -> Add8/1
  Demux3/2 -> Add1/2
  Demux2/3 -> Add3/1
  Add6/1 -> Mux2/6
  Add1/1 -> Mux2/2
  Add7/1 -> Mux2/7
  Add4/1 -> Mux2/4
  Add8/1 -> Mux2/8
  Demux2/6 -> Add6/1
  Demux3/5 -> Add5/2
  Demux2/4 -> Add4/1
  Demux2/7 -> Add7/1
  Demux2/5 -> Add5/1
  Demux3/8 -> Add8/2
  Demux3/6 -> Add6/2
  In1/1 -> Demux2/1
  Mux2/1 -> Out1/1

== system InductionHeating_bb_4/soc16/RLCsw8/add8_4 ==
  In1 : Inport
  In2 : Inport  Port=2
  Add{1..8} (8 alike) : Sum  Inputs=2
  Demux2 : Demux  Outputs=8
  Demux3 : Demux  Outputs=8
  Mux2 : Mux  Inputs=8
  Out1 : Outport
  wires:
  Mux2/1 -> Out1/1
  In1/1 -> Demux2/1
  Demux3/6 -> Add6/2
  Demux3/8 -> Add8/2
  Demux2/5 -> Add5/1
  Demux2/7 -> Add7/1
  Demux2/4 -> Add4/1
  Demux3/5 -> Add5/2
  Demux2/6 -> Add6/1
  Add8/1 -> Mux2/8
  Add4/1 -> Mux2/4
  Add7/1 -> Mux2/7
  Add1/1 -> Mux2/2
  Add6/1 -> Mux2/6
  Demux2/3 -> Add3/1
  Demux3/2 -> Add1/2
  Demux2/8 -> Add8/1
  Demux2/1 -> Add2/1
  Demux2/2 -> Add1/1
  Demux3/1 -> Add2/2
  In2/1 -> Demux3/1
  Add2/1 -> Mux2/1
  Demux3/7 -> Add7/2
  Add5/1 -> Mux2/5
  Add3/1 -> Mux2/3
  Demux3/4 -> Add4/2
  Demux3/3 -> Add3/2

== system InductionHeating_bb_4/soc16/RLCsw8/add8_5 ==
  In1 : Inport
  In2 : Inport  Port=2
  Add{1..8} (8 alike) : Sum  Inputs=2
  Demux2 : Demux  Outputs=8
  Demux3 : Demux  Outputs=8
  Mux2 : Mux  Inputs=8
  Out1 : Outport
  wires:
  Demux3/3 -> Add3/2
  Demux3/4 -> Add4/2
  Add3/1 -> Mux2/3
  Add5/1 -> Mux2/5
  Demux3/7 -> Add7/2
  Add2/1 -> Mux2/1
  In2/1 -> Demux3/1
  Demux3/1 -> Add2/2
  Demux2/2 -> Add1/1
  Demux2/1 -> Add2/1
  Demux2/8 -> Add8/1
  Demux3/2 -> Add1/2
  Demux2/3 -> Add3/1
  Add6/1 -> Mux2/6
  Add1/1 -> Mux2/2
  Add7/1 -> Mux2/7
  Add4/1 -> Mux2/4
  Add8/1 -> Mux2/8
  Demux2/6 -> Add6/1
  Demux3/5 -> Add5/2
  Demux2/4 -> Add4/1
  Demux2/7 -> Add7/1
  Demux2/5 -> Add5/1
  Demux3/8 -> Add8/2
  Demux3/6 -> Add6/2
  In1/1 -> Demux2/1
  Mux2/1 -> Out1/1

== system InductionHeating_bb_4/soc16/RLCsw8/add8_6 ==
  In1 : Inport
  In2 : Inport  Port=2
  Add{1..8} (8 alike) : Sum  Inputs=2
  Demux2 : Demux  Outputs=8
  Demux3 : Demux  Outputs=8
  Mux2 : Mux  Inputs=8
  Out1 : Outport
  wires:
  Mux2/1 -> Out1/1
  In1/1 -> Demux2/1
  Demux3/6 -> Add6/2
  Demux3/8 -> Add8/2
  Demux2/5 -> Add5/1
  Demux2/7 -> Add7/1
  Demux2/4 -> Add4/1
  Demux3/5 -> Add5/2
  Demux2/6 -> Add6/1
  Add8/1 -> Mux2/8
  Add4/1 -> Mux2/4
  Add7/1 -> Mux2/7
  Add1/1 -> Mux2/2
  Add6/1 -> Mux2/6
  Demux2/3 -> Add3/1
  Demux3/2 -> Add1/2
  Demux2/8 -> Add8/1
  Demux2/1 -> Add2/1
  Demux2/2 -> Add1/1
  Demux3/1 -> Add2/2
  In2/1 -> Demux3/1
  Add2/1 -> Mux2/1
  Demux3/7 -> Add7/2
  Add5/1 -> Mux2/5
  Add3/1 -> Mux2/3
  Demux3/4 -> Add4/2
  Demux3/3 -> Add3/2

== system InductionHeating_bb_4/soc16/RLCsw8/addsub_1 ==
  + : Inport
  - : Inport  Port=2
  Add{1..8} (8 alike) : Sum  Inputs=+-
  Demux2 : Demux  Outputs=8
  Demux3 : Demux  Outputs=8
  Mux2 : Mux  Inputs=8
  o : Outport
  wires:
  Mux2/1 -> o/1
  +/1 -> Demux2/1
  Demux3/6 -> Add6/2
  Demux3/8 -> Add8/2
  Demux2/5 -> Add5/1
  Demux2/7 -> Add7/1
  Demux2/4 -> Add4/1
  Demux3/5 -> Add5/2
  Demux2/6 -> Add6/1
  Add8/1 -> Mux2/8
  Add4/1 -> Mux2/4
  Add7/1 -> Mux2/7
  Add1/1 -> Mux2/2
  Add6/1 -> Mux2/6
  Demux2/3 -> Add3/1
  Demux3/2 -> Add1/2
  Demux2/8 -> Add8/1
  Demux2/1 -> Add2/1
  Demux2/2 -> Add1/1
  Demux3/1 -> Add2/2
  -/1 -> Demux3/1
  Add2/1 -> Mux2/1
  Demux3/7 -> Add7/2
  Add5/1 -> Mux2/5
  Add3/1 -> Mux2/3
  Demux3/4 -> Add4/2
  Demux3/3 -> Add3/2

== system InductionHeating_bb_4/soc16/RLCsw8/addsub_2 ==
  + : Inport
  - : Inport  Port=2
  Add{1..8} (8 alike) : Sum  Inputs=+-
  Demux2 : Demux  Outputs=8
  Demux3 : Demux  Outputs=8
  Mux2 : Mux  Inputs=8
  o : Outport
  wires:
  Demux3/3 -> Add3/2
  Demux3/4 -> Add4/2
  Add3/1 -> Mux2/3
  Add5/1 -> Mux2/5
  Demux3/7 -> Add7/2
  Add2/1 -> Mux2/1
  -/1 -> Demux3/1
  Demux3/1 -> Add2/2
  Demux2/2 -> Add1/1
  Demux2/1 -> Add2/1
  Demux2/8 -> Add8/1
  Demux3/2 -> Add1/2
  Demux2/3 -> Add3/1
  Add6/1 -> Mux2/6
  Add1/1 -> Mux2/2
  Add7/1 -> Mux2/7
  Add4/1 -> Mux2/4
  Add8/1 -> Mux2/8
  Demux2/6 -> Add6/1
  Demux3/5 -> Add5/2
  Demux2/4 -> Add4/1
  Demux2/7 -> Add7/1
  Demux2/5 -> Add5/1
  Demux3/8 -> Add8/2
  Demux3/6 -> Add6/2
  +/1 -> Demux2/1
  Mux2/1 -> o/1

== system InductionHeating_bb_4/soc16/RLCsw8/mmul8_1 ==
  In1 : Inport
  In2 : Inport  Port=2
  Demux2 : Demux  Outputs=8
  Demux3 : Demux  Outputs=8
  Mux2 : Mux  Inputs=8
  mult{12,15,18..19,21..22,25..26} (8 alike) : Product
  Out1 : Outport
  wires:
  Demux3/3 -> mult18/2
  Demux3/4 -> mult19/2
  mult18/1 -> Mux2/3
  mult21/1 -> Mux2/5
  Demux3/7 -> mult25/2
  mult12/1 -> Mux2/1
  In2/1 -> Demux3/1
  Demux3/1 -> mult12/2
  Demux2/2 -> mult15/1
  Demux2/1 -> mult12/1
  Demux2/8 -> mult26/1
  Demux3/2 -> mult15/2
  Demux2/3 -> mult18/1
  mult22/1 -> Mux2/6
  mult15/1 -> Mux2/2
  mult25/1 -> Mux2/7
  mult19/1 -> Mux2/4
  mult26/1 -> Mux2/8
  Demux2/6 -> mult22/1
  Demux3/5 -> mult21/2
  Demux2/4 -> mult19/1
  Demux2/7 -> mult25/1
  Demux2/5 -> mult21/1
  Demux3/8 -> mult26/2
  Demux3/6 -> mult22/2
  In1/1 -> Demux2/1
  Mux2/1 -> Out1/1

== system InductionHeating_bb_4/soc16/RLCsw8/mmul8_10 ==
  In1 : Inport
  In2 : Inport  Port=2
  Demux2 : Demux  Outputs=8
  Demux3 : Demux  Outputs=8
  Mux2 : Mux  Inputs=8
  mult{12,15,18..19,21..22,25..26} (8 alike) : Product
  Out1 : Outport
  wires:
  Demux3/3 -> mult18/2
  Demux3/4 -> mult19/2
  mult18/1 -> Mux2/3
  mult21/1 -> Mux2/5
  Demux3/7 -> mult25/2
  mult12/1 -> Mux2/1
  In2/1 -> Demux3/1
  Demux3/1 -> mult12/2
  Demux2/2 -> mult15/1
  Demux2/1 -> mult12/1
  Demux2/8 -> mult26/1
  Demux3/2 -> mult15/2
  Demux2/3 -> mult18/1
  mult22/1 -> Mux2/6
  mult15/1 -> Mux2/2
  mult25/1 -> Mux2/7
  mult19/1 -> Mux2/4
  mult26/1 -> Mux2/8
  Demux2/6 -> mult22/1
  Demux3/5 -> mult21/2
  Demux2/4 -> mult19/1
  Demux2/7 -> mult25/1
  Demux2/5 -> mult21/1
  Demux3/8 -> mult26/2
  Demux3/6 -> mult22/2
  In1/1 -> Demux2/1
  Mux2/1 -> Out1/1

== system InductionHeating_bb_4/soc16/RLCsw8/mmul8_11 ==
  In1 : Inport
  In2 : Inport  Port=2
  Demux2 : Demux  Outputs=8
  Demux3 : Demux  Outputs=8
  Mux2 : Mux  Inputs=8
  mult{12,15,18..19,21..22,25..26} (8 alike) : Product
  Out1 : Outport
  wires:
  Demux3/3 -> mult18/2
  Demux3/4 -> mult19/2
  mult18/1 -> Mux2/3
  mult21/1 -> Mux2/5
  Demux3/7 -> mult25/2
  mult12/1 -> Mux2/1
  In2/1 -> Demux3/1
  Demux3/1 -> mult12/2
  Demux2/2 -> mult15/1
  Demux2/1 -> mult12/1
  Demux2/8 -> mult26/1
  Demux3/2 -> mult15/2
  Demux2/3 -> mult18/1
  mult22/1 -> Mux2/6
  mult15/1 -> Mux2/2
  mult25/1 -> Mux2/7
  mult19/1 -> Mux2/4
  mult26/1 -> Mux2/8
  Demux2/6 -> mult22/1
  Demux3/5 -> mult21/2
  Demux2/4 -> mult19/1
  Demux2/7 -> mult25/1
  Demux2/5 -> mult21/1
  Demux3/8 -> mult26/2
  Demux3/6 -> mult22/2
  In1/1 -> Demux2/1
  Mux2/1 -> Out1/1

== system InductionHeating_bb_4/soc16/RLCsw8/mmul8_2 ==
  In1 : Inport
  In2 : Inport  Port=2
  Demux2 : Demux  Outputs=8
  Demux3 : Demux  Outputs=8
  Mux2 : Mux  Inputs=8
  mult{12,15,18..19,21..22,25..26} (8 alike) : Product
  Out1 : Outport
  wires:
  Mux2/1 -> Out1/1
  In1/1 -> Demux2/1
  Demux3/6 -> mult22/2
  Demux3/8 -> mult26/2
  Demux2/5 -> mult21/1
  Demux2/7 -> mult25/1
  Demux2/4 -> mult19/1
  Demux3/5 -> mult21/2
  Demux2/6 -> mult22/1
  mult26/1 -> Mux2/8
  mult19/1 -> Mux2/4
  mult25/1 -> Mux2/7
  mult15/1 -> Mux2/2
  mult22/1 -> Mux2/6
  Demux2/3 -> mult18/1
  Demux3/2 -> mult15/2
  Demux2/8 -> mult26/1
  Demux2/1 -> mult12/1
  Demux2/2 -> mult15/1
  Demux3/1 -> mult12/2
  In2/1 -> Demux3/1
  mult12/1 -> Mux2/1
  Demux3/7 -> mult25/2
  mult21/1 -> Mux2/5
  mult18/1 -> Mux2/3
  Demux3/4 -> mult19/2
  Demux3/3 -> mult18/2

== system InductionHeating_bb_4/soc16/RLCsw8/mmul8_3 ==
  In1 : Inport
  In2 : Inport  Port=2
  Demux2 : Demux  Outputs=8
  Demux3 : Demux  Outputs=8
  Mux2 : Mux  Inputs=8
  mult{12,15,18..19,21..22,25..26} (8 alike) : Product
  Out1 : Outport
  wires:
  Demux3/3 -> mult18/2
  Demux3/4 -> mult19/2
  mult18/1 -> Mux2/3
  mult21/1 -> Mux2/5
  Demux3/7 -> mult25/2
  mult12/1 -> Mux2/1
  In2/1 -> Demux3/1
  Demux3/1 -> mult12/2
  Demux2/2 -> mult15/1
  Demux2/1 -> mult12/1
  Demux2/8 -> mult26/1
  Demux3/2 -> mult15/2
  Demux2/3 -> mult18/1
  mult22/1 -> Mux2/6
  mult15/1 -> Mux2/2
  mult25/1 -> Mux2/7
  mult19/1 -> Mux2/4
  mult26/1 -> Mux2/8
  Demux2/6 -> mult22/1
  Demux3/5 -> mult21/2
  Demux2/4 -> mult19/1
  Demux2/7 -> mult25/1
  Demux2/5 -> mult21/1
  Demux3/8 -> mult26/2
  Demux3/6 -> mult22/2
  In1/1 -> Demux2/1
  Mux2/1 -> Out1/1

== system InductionHeating_bb_4/soc16/RLCsw8/mmul8_4 ==
  In1 : Inport
  In2 : Inport  Port=2
  Demux2 : Demux  Outputs=8
  Demux3 : Demux  Outputs=8
  Mux2 : Mux  Inputs=8
  mult{12,15,18..19,21..22,25..26} (8 alike) : Product
  Out1 : Outport
  wires:
  Mux2/1 -> Out1/1
  In1/1 -> Demux2/1
  Demux3/6 -> mult22/2
  Demux3/8 -> mult26/2
  Demux2/5 -> mult21/1
  Demux2/7 -> mult25/1
  Demux2/4 -> mult19/1
  Demux3/5 -> mult21/2
  Demux2/6 -> mult22/1
  mult26/1 -> Mux2/8
  mult19/1 -> Mux2/4
  mult25/1 -> Mux2/7
  mult15/1 -> Mux2/2
  mult22/1 -> Mux2/6
  Demux2/3 -> mult18/1
  Demux3/2 -> mult15/2
  Demux2/8 -> mult26/1
  Demux2/1 -> mult12/1
  Demux2/2 -> mult15/1
  Demux3/1 -> mult12/2
  In2/1 -> Demux3/1
  mult12/1 -> Mux2/1
  Demux3/7 -> mult25/2
  mult21/1 -> Mux2/5
  mult18/1 -> Mux2/3
  Demux3/4 -> mult19/2
  Demux3/3 -> mult18/2

== system InductionHeating_bb_4/soc16/RLCsw8/mmul8_5 ==
  In1 : Inport
  In2 : Inport  Port=2
  Demux2 : Demux  Outputs=8
  Demux3 : Demux  Outputs=8
  Mux2 : Mux  Inputs=8
  mult{12,15,18..19,21..22,25..26} (8 alike) : Product
  Out1 : Outport
  wires:
  Mux2/1 -> Out1/1
  In1/1 -> Demux2/1
  Demux3/6 -> mult22/2
  Demux3/8 -> mult26/2
  Demux2/5 -> mult21/1
  Demux2/7 -> mult25/1
  Demux2/4 -> mult19/1
  Demux3/5 -> mult21/2
  Demux2/6 -> mult22/1
  mult26/1 -> Mux2/8
  mult19/1 -> Mux2/4
  mult25/1 -> Mux2/7
  mult15/1 -> Mux2/2
  mult22/1 -> Mux2/6
  Demux2/3 -> mult18/1
  Demux3/2 -> mult15/2
  Demux2/8 -> mult26/1
  Demux2/1 -> mult12/1
  Demux2/2 -> mult15/1
  Demux3/1 -> mult12/2
  In2/1 -> Demux3/1
  mult12/1 -> Mux2/1
  Demux3/7 -> mult25/2
  mult21/1 -> Mux2/5
  mult18/1 -> Mux2/3
  Demux3/4 -> mult19/2
  Demux3/3 -> mult18/2

== system InductionHeating_bb_4/soc16/RLCsw8/mmul8_6 ==
  In1 : Inport
  In2 : Inport  Port=2
  Demux2 : Demux  Outputs=8
  Demux3 : Demux  Outputs=8
  Mux2 : Mux  Inputs=8
  mult{12,15,18..19,21..22,25..26} (8 alike) : Product
  Out1 : Outport
  wires:
  Demux3/3 -> mult18/2
  Demux3/4 -> mult19/2
  mult18/1 -> Mux2/3
  mult21/1 -> Mux2/5
  Demux3/7 -> mult25/2
  mult12/1 -> Mux2/1
  In2/1 -> Demux3/1
  Demux3/1 -> mult12/2
  Demux2/2 -> mult15/1
  Demux2/1 -> mult12/1
  Demux2/8 -> mult26/1
  Demux3/2 -> mult15/2
  Demux2/3 -> mult18/1
  mult22/1 -> Mux2/6
  mult15/1 -> Mux2/2
  mult25/1 -> Mux2/7
  mult19/1 -> Mux2/4
  mult26/1 -> Mux2/8
  Demux2/6 -> mult22/1
  Demux3/5 -> mult21/2
  Demux2/4 -> mult19/1
  Demux2/7 -> mult25/1
  Demux2/5 -> mult21/1
  Demux3/8 -> mult26/2
  Demux3/6 -> mult22/2
  In1/1 -> Demux2/1
  Mux2/1 -> Out1/1

== system InductionHeating_bb_4/soc16/RLCsw8/mmul8_7 ==
  In1 : Inport
  In2 : Inport  Port=2
  Demux2 : Demux  Outputs=8
  Demux3 : Demux  Outputs=8
  Mux2 : Mux  Inputs=8
  mult{12,15,18..19,21..22,25..26} (8 alike) : Product
  Out1 : Outport
  wires:
  Mux2/1 -> Out1/1
  In1/1 -> Demux2/1
  Demux3/6 -> mult22/2
  Demux3/8 -> mult26/2
  Demux2/5 -> mult21/1
  Demux2/7 -> mult25/1
  Demux2/4 -> mult19/1
  Demux3/5 -> mult21/2
  Demux2/6 -> mult22/1
  mult26/1 -> Mux2/8
  mult19/1 -> Mux2/4
  mult25/1 -> Mux2/7
  mult15/1 -> Mux2/2
  mult22/1 -> Mux2/6
  Demux2/3 -> mult18/1
  Demux3/2 -> mult15/2
  Demux2/8 -> mult26/1
  Demux2/1 -> mult12/1
  Demux2/2 -> mult15/1
  Demux3/1 -> mult12/2
  In2/1 -> Demux3/1
  mult12/1 -> Mux2/1
  Demux3/7 -> mult25/2
  mult21/1 -> Mux2/5
  mult18/1 -> Mux2/3
  Demux3/4 -> mult19/2
  Demux3/3 -> mult18/2
